simulink model "fangzheng"  (R2023b)
settings: Solver=ode45  StartTime=0.0  StopTime=1.5  RelTol=1e-6
InitFcn:
  | Rf=0.05;Lf=2e-3;Cf=50e-6;fn=50;w0=2*fn*pi;
  | UB=3e3;SB=1e6;IB=SB/(sqrt(3)*UB);
  | Xf=Lf*w0;Z=sqrt((Rf^2+Xf^2));
  | J=3;D=2e4/w0*0;kf=0.9e4/w0;
  | K=230*380/Xf;
  | P=10;I=12e3;
  | Jw=8e4;
  | Pi=1;Pp=0;P2 =1000;
  | U5=30;
  | U7=15;
undefined symbols (not defined in the file): sigbuilder_block
libraries: slpidlib x5, spsThreePhaseSeriesRLCBranchLib x4, spsThreePhaseBreakerLib x3, spsabctodq0Lib x3, simulink x3, spsThreePhaseVIMeasurementLib x3, spsControlledVoltageSourceLib x3, spsThreePhaseSeriesRLCLoadLib x2, spsDCVoltageSourceLib x1, spsUniversalBridgeLib x1, spsPWMGenerator2LevelLib x1, spsdq0toabcLib x1
settings Model: SimulationMode=accelerator  Creator=lenovo  LastModifiedBy=Administrator
settings SolverCC: ZeroCrossAlgorithm=Adaptive  AlgebraicLoopSolver=TrustRegion
settings DataIOCC: SaveFormat=StructureWithTime  ReturnWorkspaceOutputs=off
settings OptimizationCC: DefaultParameterBehavior=Inlined  EnhancedBackFolding=on  PassReuseOutputArgsAs=Individual arguments  ZeroExternalMemoryAtStartup=off  ZeroInternalMemoryAtStartup=off  AccelVerboseBuild=on  OptimizeBlockOrder=speed  DifferentSizesBufferReuse=on  OptimizationCustomize=off  EfficientTunableParamExpr=on
settings DebuggingCC: IgnoredZcDiagnostic=none  ParameterTunabilityLossMsg=error  UnconnectedInputMsg=warning  UnconnectedOutputMsg=warning  UnconnectedLineMsg=warning  ArithmeticOperatorsInVariantConditions=warning
settings ModelReferenceCC: EnableRefExpFcnMdlSchedulingChecks=on
settings SFSimCC: MATLABDynamicMemAlloc=off  CustomCodeUndefinedFunction=UseInterfaceOnly
settings RTWCC: Description=Embedded Coder  SystemTargetFile=ert.tlc  TemplateMakefile=ert_default_tmf
settings CodeAppCC: ForceParamTrailComments=on  IgnoreCustomStorageClasses=off  OperatorAnnotations=on  SimulinkDataObjDesc=on  SFDataObjDesc=on  InsertBlockDesc=on
settings ERTTargetCC: TargetLangStandard=C99 (ISO)  GenerateSampleERTMain=on  InlinedParameterPlacement=NonHierarchical  ERTCustomFileTemplate=example_file_process.tlc

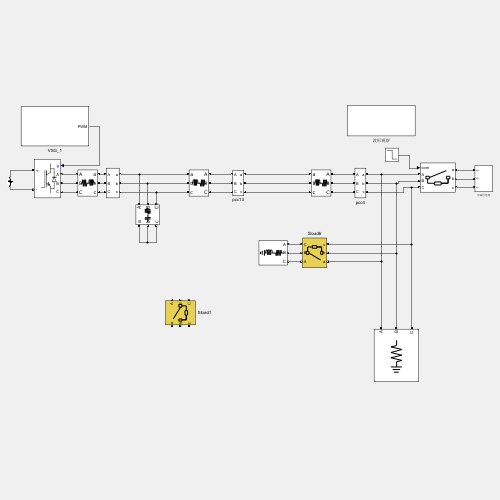
[thumbnail: Simulink's stored preview of the top-level diagram]
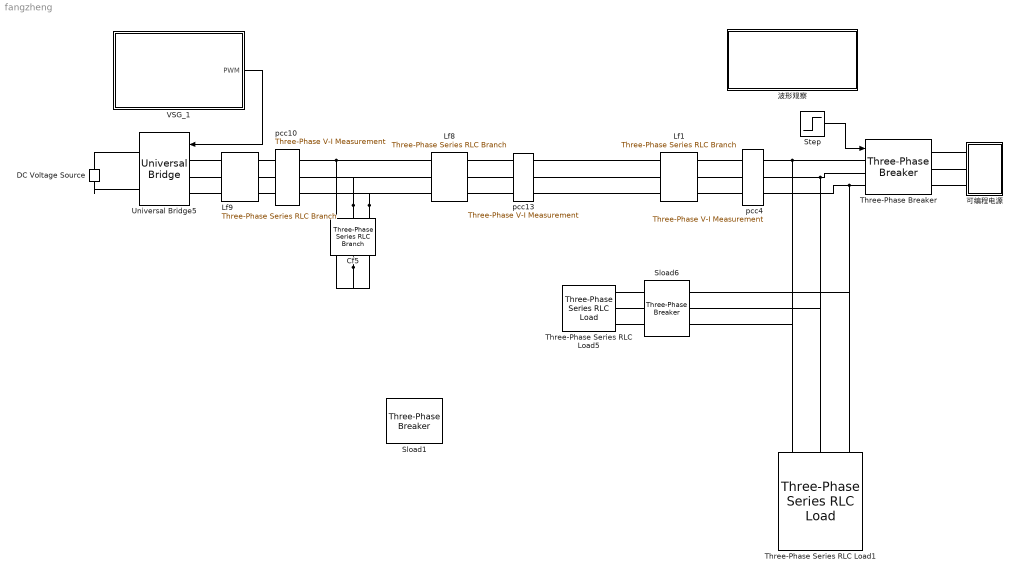
== system fangzheng ==
  " Lf1" : spsThreePhaseSeriesRLCBranchLib/Three-Phase Series RLC Branch  LConnTagsString=A|B|C  RConnTagsString=A|B|C  BranchType=RL  Resistance=0.1  Inductance=0.0002  Capacitance=0  Measurements=None
  " Lf8" : spsThreePhaseSeriesRLCBranchLib/Three-Phase Series RLC Branch  LConnTagsString=A|B|C  RConnTagsString=A|B|C  BranchType=RL  Resistance=0.02  Inductance=0.004  Capacitance=0  Measurements=None
  " Lf9" : spsThreePhaseSeriesRLCBranchLib/Three-Phase Series RLC Branch  LConnTagsString=A|B|C  RConnTagsString=A|B|C  BranchType=RL  Resistance=0.1  Inductance=0.005  Capacitance=0  Measurements=None
  Cf5 : spsThreePhaseSeriesRLCBranchLib/Three-Phase Series RLC Branch  LConnTagsString=A|B|C  RConnTagsString=A|B|C  BranchType=RC  Resistance=0.5  Inductance=4e-3  Capacitance=3e-5  Measurements=None
  DC Voltage Source : spsDCVoltageSourceLib/DC Voltage Source  Amplitude=800  Measurements=None
  Sload1 : spsThreePhaseBreakerLib/Three-Phase Breaker  InitialState=open  SwitchA=on  SwitchB=on  SwitchC=on  SwitchTimes=[1.0]  External=off  BreakerResistance=0.0001  SnubberResistance=1e6  SnubberCapacitance=inf  Measurements=None
  Sload6 : spsThreePhaseBreakerLib/Three-Phase Breaker  InitialState=open  SwitchA=on  SwitchB=on  SwitchC=on  SwitchTimes=[1.2]  External=off  BreakerResistance=0.0001  SnubberResistance=1e6  SnubberCapacitance=inf  Measurements=None
  Step : Step  Before=1  After=0  SampleTime=0
  Three-Phase Series RLC Load1 : spsThreePhaseSeriesRLCLoadLib/Three-Phase Series RLC Load  LConnTagsString=A|B|C  Configuration=Y (grounded)  NominalVoltage=380  Vabc=[1e3 1e3 1e3]  Vabcp=[1e3 1e3 1e3]  NominalFrequency=50  UnbalancedPower=off  ActivePower=15e3  InductivePower=0  CapacitivePower=0  Pabc=[10e3 9e3 11e3]  QLabc=[100 90 110]  QCabc=[100 90 110]  Pabcp=[10e3 9e3 11e3]  QLabcp=[100 90 110]  QCabcp=[100 90 110]  Measurements=None  LoadType=constant Z
  Three-Phase Series RLC Load5 : spsThreePhaseSeriesRLCLoadLib/Three-Phase Series RLC Load  LConnTagsString=A|B|C  Configuration=Y (grounded)  NominalVoltage=380  Vabc=[1e3 1e3 1e3]  Vabcp=[1e3 1e3 1e3]  NominalFrequency=50  UnbalancedPower=off  ActivePower=15e3  InductivePower=6e3  CapacitivePower=0  Pabc=[10e3 9e3 11e3]  QLabc=[100 90 110]  QCabc=[100 90 110]  Pabcp=[10e3 9e3 11e3]  QLabcp=[100 90 110]  QCabcp=[100 90 110]  Measurements=None  LoadType=constant Z
  Three-Phase Breaker : spsThreePhaseBreakerLib/Three-Phase Breaker  InitialState=open  SwitchA=on  SwitchB=on  SwitchC=on  SwitchTimes="[1/60  5/60]"  External=on  BreakerResistance=0.01  SnubberResistance=1e6  SnubberCapacitance=inf  Measurements=None
  Universal Bridge5 : spsUniversalBridgeLib/Universal Bridge  Arms=3  SnubberResistance=1e5  SnubberCapacitance=inf  Device=IGBT / Diodes  Ron=1e-5  Lon=0  ForwardVoltages=[0.05 0.05]  ForwardVoltage=0  GTOparameters=[ 10e-6 , 20e-6 ]  IGBTparameters=[ 1e-6 , 2e-6 ]  Measurements=None  Measurements_2=None  converterType=Rectifier
  VSG_1 : Subsystem
  pcc10 : spsThreePhaseVIMeasurementLib/Three-Phase V-I Measurement  VoltageMeasurement=phase-to-ground  SetLabelV=on  LabelV=Vo_1  Vpu=off  VpuLL=off  CurrentMeasurement=yes  SetLabelI=on  LabelI=IL_1  Ipu=off  Pbase=1e6  Vbase=6.6e3/sqrt(3)  OutputType=Magnitude  PhasorSimulation=off  PSBequivalent=0
  pcc13 : spsThreePhaseVIMeasurementLib/Three-Phase V-I Measurement  VoltageMeasurement=phase-to-ground  SetLabelV=on  LabelV=Vabc_pcc_1  Vpu=off  VpuLL=off  CurrentMeasurement=yes  SetLabelI=on  LabelI=Iabc_pcc_1  Ipu=off  Pbase=1e6  Vbase=6.6e3/sqrt(3)  OutputType=Magnitude  PhasorSimulation=off  PSBequivalent=0
  pcc4 : spsThreePhaseVIMeasurementLib/Three-Phase V-I Measurement  VoltageMeasurement=phase-to-ground  SetLabelV=on  LabelV=Vg  Vpu=off  VpuLL=off  CurrentMeasurement=yes  SetLabelI=on  LabelI=Ig  Ipu=off  Pbase=1e6  Vbase=6.6e3/sqrt(3)  OutputType=Magnitude  PhasorSimulation=off  PSBequivalent=0
  可编程电源 : Subsystem
  波形观察 : Subsystem
  wires:
  VSG_1/1(PWM) -> Universal Bridge5/1
  Step/1 -> Three-Phase Breaker/1
  connections:
  Cf5/RConn2 -- Cf5/RConn3 -- Cf5/RConn1
  " Lf9"/LConn3 -- Universal Bridge5/LConn3
  " Lf9"/LConn1 -- Universal Bridge5/LConn1
  " Lf9"/LConn2 -- Universal Bridge5/LConn2
  " Lf8"/RConn1 -- pcc10/RConn1 -- Cf5/LConn1
  Cf5/LConn3 -- pcc10/RConn3 -- " Lf8"/RConn3
  Cf5/LConn2 -- pcc10/RConn2 -- " Lf8"/RConn2
  " Lf1"/LConn2 -- pcc4/LConn2
  pcc4/LConn3 -- " Lf1"/LConn3
  pcc4/LConn1 -- " Lf1"/LConn1
  " Lf1"/RConn1 -- pcc13/RConn1
  " Lf1"/RConn2 -- pcc13/RConn2
  " Lf1"/RConn3 -- pcc13/RConn3
  " Lf8"/LConn1 -- pcc13/LConn1
  " Lf8"/LConn2 -- pcc13/LConn2
  " Lf8"/LConn3 -- pcc13/LConn3
  DC Voltage Source/RConn1 -- Universal Bridge5/RConn1
  DC Voltage Source/LConn1 -- Universal Bridge5/RConn2
  " Lf9"/RConn1 -- pcc10/LConn1
  " Lf9"/RConn2 -- pcc10/LConn2
  " Lf9"/RConn3 -- pcc10/LConn3
  Three-Phase Breaker/RConn1 -- 可编程电源/RConn1
  Three-Phase Breaker/RConn2 -- 可编程电源/RConn2
  Three-Phase Breaker/RConn3 -- 可编程电源/RConn3
  Sload6/LConn3 -- Three-Phase Series RLC Load5/LConn1
  Sload6/LConn2 -- Three-Phase Series RLC Load5/LConn2
  Sload6/LConn1 -- Three-Phase Series RLC Load5/LConn3
  Three-Phase Breaker/LConn1 -- Three-Phase Series RLC Load1/LConn1 -- Sload6/RConn1 -- pcc4/RConn1
  pcc4/RConn2 -- Three-Phase Series RLC Load1/LConn2 -- Sload6/RConn2 -- Three-Phase Breaker/LConn2
  Three-Phase Breaker/LConn3 -- Sload6/RConn3 -- Three-Phase Series RLC Load1/LConn3 -- pcc4/RConn3

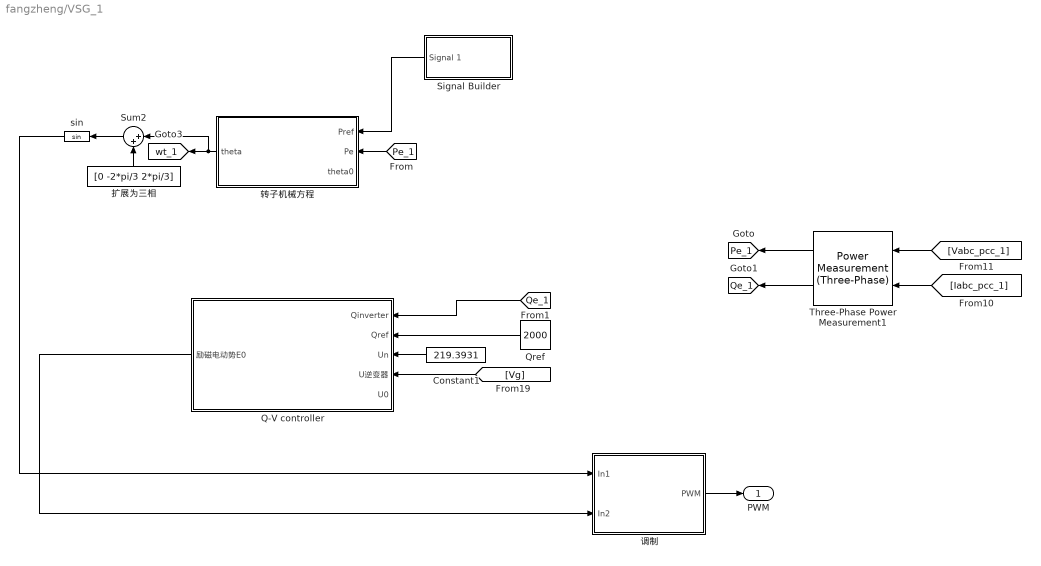
== system fangzheng/VSG_1 ==
  " 调制" : Subsystem
  Constant1 : Constant  Value=219.3931
  Q-V controller : Subsystem
  Qref : Constant  Value=2000
  Signal Builder : Subsystem  Tag=STV Subsys  LoadFcn=sigbuilder_block('load');  StartFcn=sigbuilder_block('start');  StopFcn=sigbuilder_block('stop');  ClipboardFcn=sigbuilder_block('clipboard');  mask(Sigbuilder block){tuvar=[0:10]}
      mask help: Simulink:masks:SigbuilderBlock_MD
      mask init:
      | if ~strcmp(get_param(bdroot(gcbh),'SimulationStatus'),'stopped') tuvar = sigbuilder_block('maskInit'); end
      settings: CopyFcn=sigbuilder_block('copy');  DeleteFcn=sigbuilder_block('delete');  ModelCloseFcn=sigbuilder_block('modelClose');  PreSaveFcn=sigbuilder_block('preSave');  PauseFcn=sigbuilder_block('pause');  ContinueFcn=sigbuilder_block('continue');  NameChangeFcn=sigbuilder_block('namechange');  OpenFcn=sigbuilder_block('open',[4.875 36 1430.25 685.125 ]);  CloseFcn=sigbuilder_block('close');
      mask Display: plot(0, 0, 100, 100,[2, 2, 32, 32, 2], [68, 8, 8, 68, 68],[32, 2], [38, 38], [32, 19, 2],[53, 60, 44], [32, 17, 17, 2],[16, 16, 31, 31]);txt = getActiveGroup(gcbh);text(2, 100, txt,'verticalAlignment', 'top');
  Sum2 : Sum  Inputs=|++
  Three-Phase Power Measurement1 : eePowerMeasurement/Power Measurement (Three-Phase)  LabelModeActiveChoice=Continuous  F=50  K=[1]  Seq=Positive  Ts=0
  sin : Trigonometry
  扩展为三相 : Constant  Value=[0 -2*pi/3 2*pi/3]
  转子机械方程 : Subsystem
  PWM : Outport
  tag scope: Pe_1=global, Qe_1=global, wt_1=global
  wires:
  扩展为三相/1 -> Sum2/2
  Three-Phase Power Measurement1/1 -> [Pe_1]
  [Iabc_pcc_1] -> Three-Phase Power Measurement1/2
  Qref/1 -> Q-V controller/2(Qref)
  [Vg] -> Q-V controller/4(U逆变器)
  [Vabc_pcc_1] -> Three-Phase Power Measurement1/1
  转子机械方程/1(theta) -> Sum2/1, [wt_1]
  Three-Phase Power Measurement1/2 -> [Qe_1]
  Constant1/1 -> Q-V controller/3(Un)
  Sum2/1 -> sin/1
  Signal Builder/1(Signal 1) -> 转子机械方程/1(Pref)
  sin/1 -> " 调制"/1(In1)
  Q-V controller/1(励磁电动势E0) -> " 调制"/2(In2)
  " 调制"/1(PWM) -> PWM/1
  [Pe_1] -> 转子机械方程/2(Pe)
  [Qe_1] -> Q-V controller/1(Qinverter)

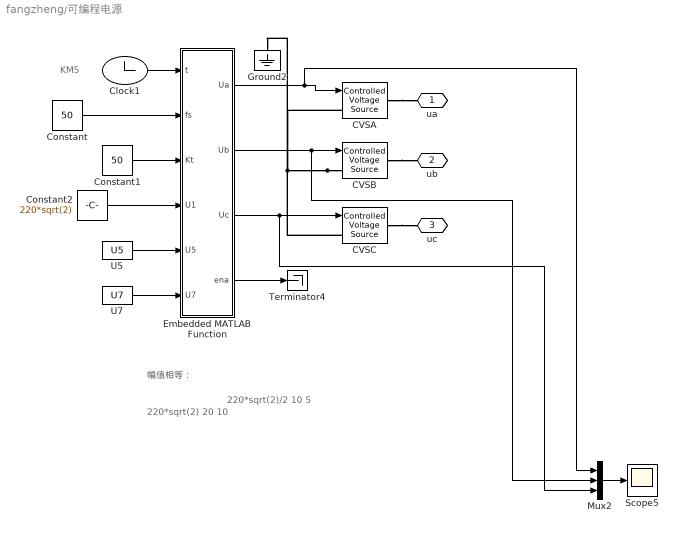
== system fangzheng/可编程电源 ==
  note: KM5
  note: 幅值相等：
  note: 220*sqrt(2)
      | 20
      | 10
  note: 220*sqrt(2)/2
      | 10
      | 5
  CVSA : spsControlledVoltageSourceLib/Controlled Voltage Source  Initialize=on  Source_Type=AC  Amplitude=0  Phase=0  Frequency=0  Measurements=None
  CVSB : spsControlledVoltageSourceLib/Controlled Voltage Source  Initialize=on  Source_Type=AC  Amplitude=0  Phase=0  Frequency=0  Measurements=None
  CVSC : spsControlledVoltageSourceLib/Controlled Voltage Source  Initialize=on  Source_Type=AC  Amplitude=0  Phase=0  Frequency=0  Measurements=None
  Clock1 : Clock
  Constant : Constant  Value=50
  Constant1 : Constant  Value=50
  Constant2 : Constant  Value=220*sqrt(2)
  Embedded MATLAB Function : MATLAB Function  TreatAsAtomicUnit=on
  Ground2 : spsGroundLib/Ground  LConnTagsString=a
  Mux2 : Mux  Inputs=3
  Scope5 : Scope
  Terminator4 : Terminator
  U5 : Constant  Value=U5
  U7 : Constant  Value=U7
  ua : PMIOPort  Side=Right
  ub : PMIOPort  Port=2  Side=Right
  uc : PMIOPort  Port=3  Side=Right
  wires:
  Clock1/1 -> Embedded MATLAB Function/1(t)
  U5/1 -> Embedded MATLAB Function/5(U5)
  Embedded MATLAB Function/3(Uc) -> Mux2/3, CVSC/1
  U7/1 -> Embedded MATLAB Function/6(U7)
  Embedded MATLAB Function/4(ena) -> Terminator4/1
  Constant1/1 -> Embedded MATLAB Function/3(Kt)
  Constant/1 -> Embedded MATLAB Function/2(fs)
  Embedded MATLAB Function/2(Ub) -> Mux2/2, CVSB/1
  Mux2/1 -> Scope5/1
  Embedded MATLAB Function/1(Ua) -> Mux2/1, CVSA/1
  Constant2/1 -> Embedded MATLAB Function/4(U1)
  connections:
  CVSC/RConn1 -- uc/RConn1
  CVSB/RConn1 -- ub/RConn1
  CVSA/RConn1 -- ua/RConn1
  CVSB/LConn1 -- Ground2/LConn1 -- CVSA/LConn1 -- CVSC/LConn1

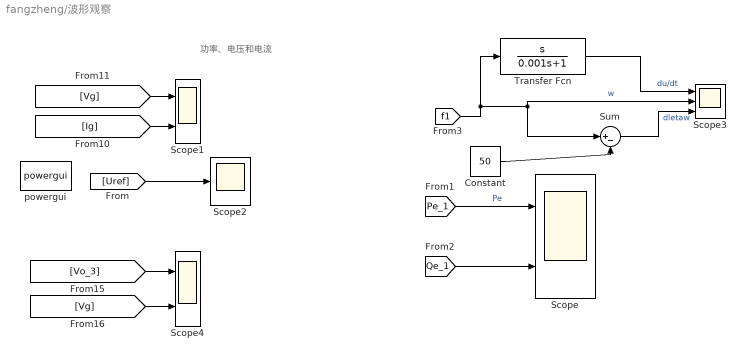
== system fangzheng/波形观察 ==
  note: 功率、电压和电流
  Constant : Constant  Value=50
  Scope : Scope  NumInputPorts=2
  Scope1 : Scope  NumInputPorts=2
  Scope2 : Scope
  Scope3 : Scope  NumInputPorts=3
  Scope4 : Scope  NumInputPorts=2
  Sum : Sum  Inputs=|+-
  Transfer Fcn : TransferFcn  Numerator=[1 0]  Denominator=[0.001 1]
  powergui : sps_lib/powergui  Priority=1  SimulationMode=Discrete  SampleTime=1e-6  frequency=60  Iterations=50  frequencyindice=0  Pbase=100e6  ErrMax=1e-4  UnitsV=kV  UnitsW=MW  buscounter=0  FunctionMessages=off  echomessages=off  EnableUseOfTLC=off  CurrentSourceSwitches=off  DisableSnubberDevices=off  DisableRonSwitches=off  DisableVfSwitches=off  DisplayEquations=off  AutomaticDiscreteSolvers=off  SolverType=Tustin/Backward Euler (TBE)  Interpol=off  ExternalGateDelay=off  methode=off  Ts=100  x0status=blocks  SPID=on  SwTol=0  HookPort=off  NonlinearTolerance=1e-4  nMaxIteration=100  ContinueOnMaxIteration=off  RestoreLinks=warning  ResistiveCurrentMeasurement=off  Frange=[0:2:500]  Ylog=off  Xlog=on  ShowGrid=off  save=off  variable=ZData  structure=logsout  ZoomFFT=off  StartTime=0.5  cycles=10  DisplayStyle=1  fundamental=50  FreqAxis=off  MaxFrequency=1000  frequencyindicesteady=1  RmsSteady=1  display=off
  wires:
  [Vg] -> Scope1/1
  [Qe_1] -> Scope/2
  [Pe_1] -> Scope/1  "Pe"
  [Ig] -> Scope1/2
  [Uref] -> Scope2/1
  [f1] -> Sum/1, Scope3/2, Transfer Fcn/1  "w"
  [Vo_3] -> Scope4/1
  [Vg] -> Scope4/2
  Transfer Fcn/1 -> Scope3/1  "du/dt"
  Constant/1 -> Sum/2
  Sum/1 -> Scope3/3  "dletaw"

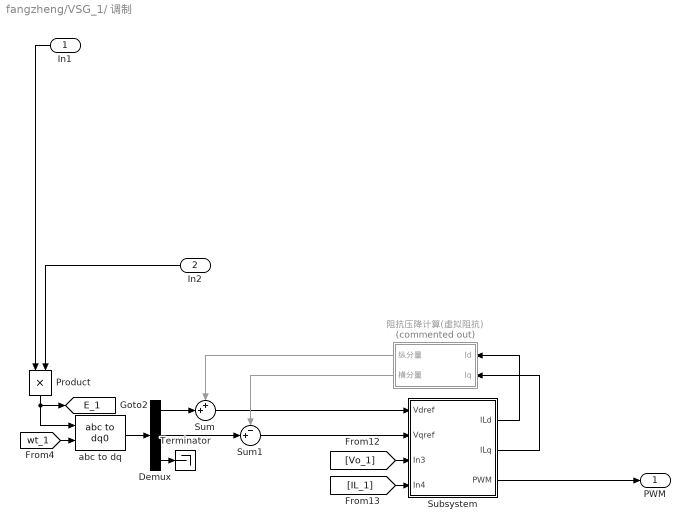
== system fangzheng/VSG_1/ 调制 ==
  In1 : Inport
  In2 : Inport  Port=2
  Demux : Demux  Outputs=3
  Product : Product
  Subsystem : Subsystem
  Sum : Sum  Inputs=++|
  Sum1 : Sum  Inputs=-+|
  Terminator : Terminator
  abc to dq : spsabctodq0Lib/abc to dq0  Alignment=90 degrees behind phase A axis
  阻抗压降计算(虚拟阻抗) : Subsystem  Commented=on
  PWM : Outport
  tag scope: E_1=global
  wires:
  [Vo_1] -> Subsystem/3(In3)
  Demux/2 -> Sum1/2
  Sum/1 -> Subsystem/1(Vdref)
  [IL_1] -> Subsystem/4(In4)
  abc to dq/1 -> Demux/1
  Subsystem/1(ILd) -> 阻抗压降计算(虚拟阻抗)/1(Id)
  Demux/1 -> Sum/2
  阻抗压降计算(虚拟阻抗)/1(纵分量) -> Sum/1
  Demux/3 -> Terminator/1
  Sum1/1 -> Subsystem/2(Vqref)
  Product/1 -> [E_1], abc to dq/1
  Subsystem/2(ILq) -> 阻抗压降计算(虚拟阻抗)/2(Iq)
  阻抗压降计算(虚拟阻抗)/2(横分量) -> Sum1/1
  Subsystem/3(PWM) -> PWM/1
  [wt_1] -> abc to dq/2
  In1/1 -> Product/1
  In2/1 -> Product/2

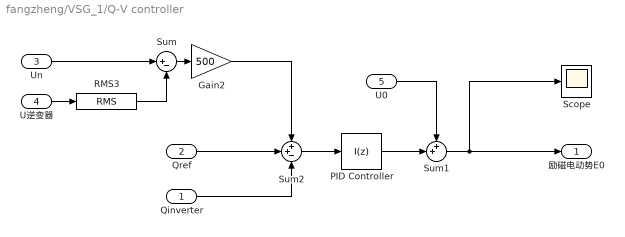
== system fangzheng/VSG_1/Q-V controller ==
  Qinverter : Inport
  Qref : Inport  Port=2
  Un : Inport  Port=3
  U逆变器 : Inport  Port=4
  U0 : Inport  Port=5
  Gain2 : Gain  Gain=500
  PID Controller : slpidlib/PID Controller  Controller=I  Form=Parallel  TimeDomain=Discrete-time  UseExternalTs=off  SampleTime=-1  IntegratorMethod=Forward Euler  FilterMethod=Forward Euler  ControllerParametersSource=internal  P=0.0000001  I=1.1547e-5*5  UseKiTs=off  D=0  N=100  UseFilter=on  TunerSelectOption=Transfer Function Based (PID Tuner App)  InitialConditionSource=internal  InitialConditionForIntegrator=0  InitialConditionForFilter=0  DifferentiatorICPrevScaledInput=0  ExternalReset=none  TrackingMode=off  Kt=1  LimitOutput=off  SatLimitsSource=internal  UpperSaturationLimit=inf  LowerSaturationLimit=-inf  LinearizeAsGain=on  AntiWindupMode=none  Kb=1  LimitIntegrator=off  UpperIntegratorSaturationLimit=inf  LowerIntegratorSaturationLimit=-inf  POutMin=[]  POutMax=[]  IOutMin=[]  IOutMax=[]  DOutMin=[]  DOutMax=[]  NOutMin=[]  NOutMax=[]  SumOutMin=[]  SumOutMax=[]  SaturationOutMin=[]  SaturationOutMax=[]  PParamMin=[]  PParamMax=[]  IParamMin=[]  IParamMax=[]  DParamMin=[]  DParamMax=[]  NParamMin=[]  NParamMax=[]  KbParamMin=[]  KbParamMax=[]  KtParamMin=[]  KtParamMax=[]  KbOutMin=[]  KbOutMax=[]  KtOutMin=[]  KtOutMax=[]  IntegratorOutMin=[]  IntegratorOutMax=[]  FilterOutMin=[]  FilterOutMax=[]  SumI1OutMin=[]  SumI1OutMax=[]  SumI2OutMin=[]  SumI2OutMax=[]  SumI3OutMin=[]  SumI3OutMax=[]  SumI4OutMin=[]  SumI4OutMax=[]  SumDOutMin=[]  SumDOutMax=[]  DifferentiatorOutMin=[]  DifferentiatorOutMax=[]  FilterDiffOutCoefMin=[]  FilterDiffOutCoefMax=[]  ReciprocalOutMin=[]  ReciprocalOutMax=[]  SumDenOutMin=[]  SumDenOutMax=[]  SumNumOutMin=[]  SumNumOutMax=[]  DivideOutMin=[]  DivideOutMax=[]  UdiffTsProdOutMin=[]  UdiffTsProdOutMax=[]  NTsProdOutMin=[]  NTsProdOutMax=[]  UintegralTsProdOutMin=[]  UintegralTsProdOutMax=[]  UngainTsProdOutMin=[]  UngainTsProdOutMax=[]  ClampingZeroOutDataTypeStr=Inherit: Inherit via back propagation  ClampingZeroOutMin=[]  ClampingZeroOutMax=[]  FilterDenConstantOutDataTypeStr=Inherit: Inherit via back propagation  FilterDenConstantOutMin=[]  FilterDenConstantOutMax=[]  PCopyOutDataTypeStr=Inherit: Inherit via back propagation  PCopyOutMin=[]  PCopyOutMax=[]  NCopyOutDataTypeStr=Inherit: Inherit via back propagation  NCopyOutMin=[]  NCopyOutMax=[]  IntegratorContinuousStateAttributes=''  IntegratorStateMustResolveToSignalObject=off  IntegratorRTWStateStorageClass=Auto  FilterContinuousStateAttributes=''  FilterStateMustResolveToSignalObject=off  FilterRTWStateStorageClass=Auto  ParallelPVariant=Disabled  IdealPVariant=Disabled  IVariant=InternalParameters  DVariant=Disabled  IntegratorVariant=Discrete  SatVariant=Disabled  AWVariant=Passthrough  PCopyVariant=Disabled  TRVariant=Disabled  FdbkBlocksVariant=Forward  IdealPFdbkVariant=Disabled  SatFdbkVariant=Disabled  DerivativeFilterVariant=Disabled  NVariant=Disabled  NCopyVariant=Disabled_SignalSpec  FilterICVariant=Disabled  IntegratorICVariant=InternalICs  ExternalResetVariant=Disabled  TRSumVariant=Passthrough  SumFdbkVariant=Disabled  SumVariant=Passthrough_I  TsampFilterVariant=InternalTs  TsampNgainVariant=Passthrough  TsampIntegralVariant=Disabled_SignalSpec  ExternalSaturationOutDataTypeStr=Inherit: Same as second input
  RMS3 : dspstat3/RMS  run=off  directionMode=Each column  dimension=1  InputProcessing=Columns as channels (frame based)  reset_popup=None
  Scope : Scope
  Sum : Sum  Inputs=|+-
  Sum1 : Sum  Inputs=++|
  Sum2 : Sum  Inputs=++-
  励磁电动势E0 : Outport
  wires:
  Qinverter/1 -> Sum2/3
  Qref/1 -> Sum2/2
  Un/1 -> Sum/1
  U逆变器/1 -> RMS3/1
  Gain2/1 -> Sum2/1
  Sum/1 -> Gain2/1
  RMS3/1 -> Sum/2
  Sum2/1 -> PID Controller/1
  U0/1 -> Sum1/1
  Sum1/1 -> 励磁电动势E0/1, Scope/1
  PID Controller/1 -> Sum1/2

== system fangzheng/VSG_1/Signal Builder ==
  Demux : Demux  Tag=STV Demux  Outputs=1
      settings: DisplayOption=none
  FromWs : FromWorkspace  Tag=STV FromWs  VariableName=tuvar
      SigBuilderData=|
      | common.afterFinalStr = 'Extrapolate'
      | common.sampleTime = 0
      | dataSet.timeRange = [0 10]
      | dataSet.name = 'Group 1'
      | sbobj.Groups.Name = 'Group 1'
      | sbobj.Groups.Signals.Name = 'Signal 1'
      | sbobj.Groups.Signals.XData = [0 0.5 0.5 2 2 3.93 3.93 6 6 10]
      | sbobj.Groups.Signals.YData = [0 0 15700 15700 30100 30100 0 0 -0.2 -0.2]
  Signal 1 : Outport  Tag=STV Outport  VectorParamsAs1DForOutWhenUnconnected=off
  wires:
  FromWs/1 -> Demux/1
  Demux/1 -> Signal 1/1

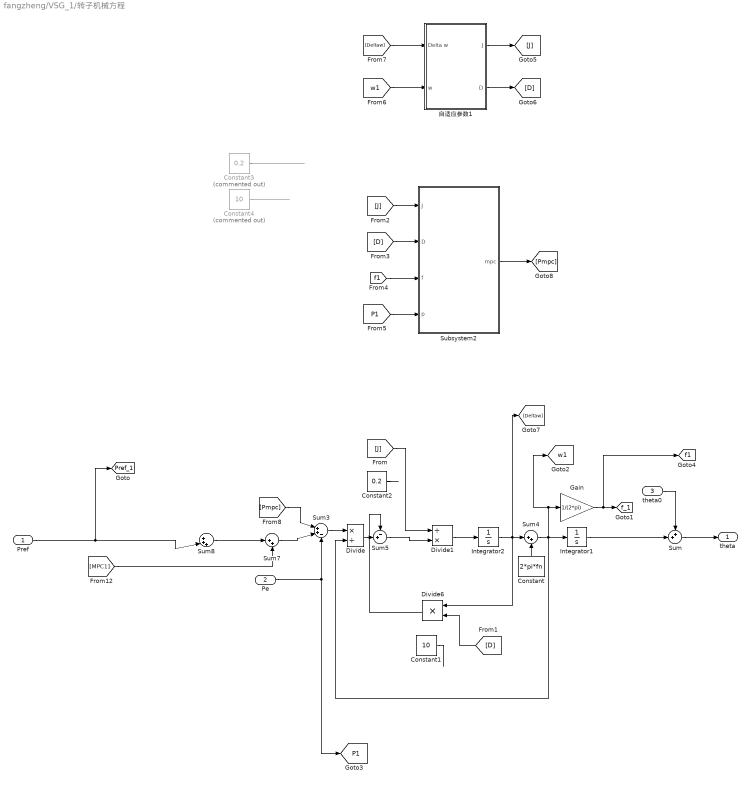
== system fangzheng/VSG_1/转子机械方程 ==
  Pref : Inport
  Pe : Inport  Port=2
  theta0 : Inport  Port=3
  Constant : Constant  Value=2*pi*fn
  Constant1 : Constant  Value=10
  Constant2 : Constant  Value=0.2
  Constant3 : Constant  Commented=on  Value=0.2
  Constant4 : Constant  Commented=on  Value=10
  Divide : Product  Inputs=*/
  Divide1 : Product  Inputs=/*
  Divide6 : Product  Inputs=**
  Gain : Gain  Gain=1/(2*pi)
  Integrator1 : Integrator
  Integrator2 : Integrator
  Subsystem2 : Subsystem
  Sum : Sum  Inputs=++|
  Sum3 : Sum  Inputs=|++-
  Sum4 : Sum  Inputs=|++
  Sum5 : Sum  Inputs=-+|
  Sum7 : Sum  Inputs=|++
  Sum8 : Sum  Inputs=|+++
  自适应参数1 : Subsystem
  theta : Outport
  tag scope: P1=global, Pref_1=global, f1=global, f_1=global, w1=global
  wires:
  Constant/1 -> Sum4/2
  Divide/1 -> Sum5/2
  Sum3/1 -> Divide/1
  Divide1/1 -> Integrator2/1
  theta0/1 -> Sum/1
  Sum/1 -> theta/1
  Integrator1/1 -> Sum/2
  Subsystem2/1(mpc) -> [Pmpc]
  Pref/1 -> Sum8/2, [Pref_1]
  Sum8/1 -> Sum7/1
  Gain/1 -> [f1], [f_1]
  Sum7/1 -> Sum3/2
  Pe/1 -> Sum3/3, [P1]
  [MPC1] -> Sum7/2
  Divide6/1 -> Sum5/1
  [D] -> Divide6/2
  Sum5/1 -> Divide1/2
  Constant2/1 -> ?
  自适应参数1/2(D) -> [D]
  Sum4/1 -> Divide/2, Integrator1/1, [w1], Gain/1
  Integrator2/1 -> [Deltaw], Divide6/1, Sum4/1
  自适应参数1/1(J) -> [J]
  Constant3/1 -> ?
  Constant4/1 -> ?
  [J] -> Divide1/1
  [J] -> Subsystem2/1(J)
  [D] -> Subsystem2/2(D)
  Constant1/1 -> ?
  [f1] -> Subsystem2/3(f)
  [P1] -> Subsystem2/4(p)
  [w1] -> 自适应参数1/2(w)
  [Deltaw] -> 自适应参数1/1(Delta w)
  [Pmpc] -> Sum3/1

== system fangzheng/VSG_1/ 调制/Subsystem ==
  Vdref : Inport
  Vqref : Inport  Port=2
  In3 : Inport  Port=3
  In4 : Inport  Port=4
  Gain5 : Gain  Gain=1/(SB/(sqrt(3)*UB))
  Gain6 : Gain  Gain=sqrt(3)/UB
  abc2dq0 : Subsystem
  电压电流双闭环 : Subsystem
  ILd : Outport
  ILq : Outport  Port=2
  PWM : Outport  Port=3
  wires:
  Vqref/1 -> 电压电流双闭环/2(Vqref)
  In4/1 -> Gain5/1
  abc2dq0/1(Vd) -> 电压电流双闭环/3(Vd)
  abc2dq0/2(Vq) -> 电压电流双闭环/4(Vq)
  abc2dq0/3(ILd) -> 电压电流双闭环/5(ILd), ILd/1
  Gain5/1 -> abc2dq0/2(Iabc)
  Gain6/1 -> abc2dq0/1(Vabc)
  abc2dq0/4(ILq) -> 电压电流双闭环/6(ILq), ILq/1
  电压电流双闭环/1(PWM) -> PWM/1
  Vdref/1 -> 电压电流双闭环/1(Vdref)
  In3/1 -> Gain6/1

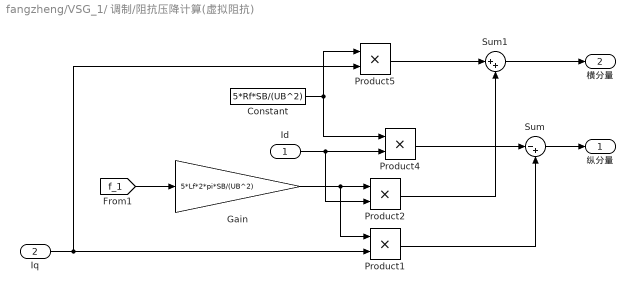
== system fangzheng/VSG_1/ 调制/阻抗压降计算(虚拟阻抗) ==
  Id : Inport
  Iq : Inport  Port=2
  Constant : Constant  Value=5*Rf*SB/(UB^2)
  Gain : Gain  Gain=5*Lf*2*pi*SB/(UB^2)
  Product{1..2,4..5} (4 alike) : Product
  Sum : Sum  Inputs=|-+
  Sum1 : Sum  Inputs=|++
  纵分量 : Outport
  横分量 : Outport  Port=2
  wires:
  Product2/1 -> Sum1/2
  Sum1/1 -> 横分量/1
  Product5/1 -> Sum1/1
  Sum/1 -> 纵分量/1
  Product1/1 -> Sum/2
  Product4/1 -> Sum/1
  Gain/1 -> Product1/1, Product2/1
  Iq/1 -> Product5/2, Product1/2
  [f_1] -> Gain/1
  Constant/1 -> Product5/1, Product4/1
  Id/1 -> Product2/2, Product4/2

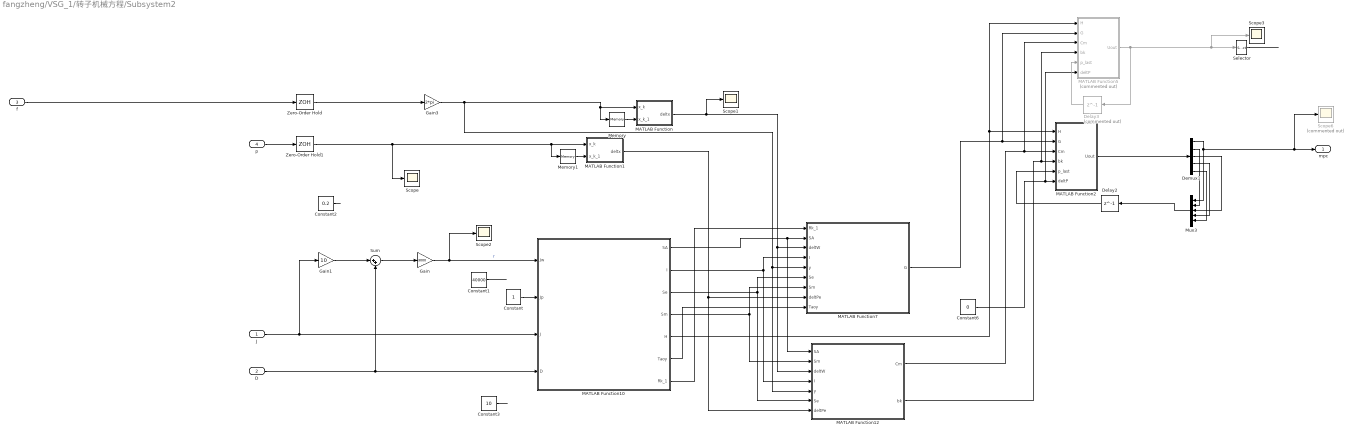
== system fangzheng/VSG_1/转子机械方程/Subsystem2 ==
  J : Inport
  D : Inport  Port=2
  f : Inport  Port=3
  p : Inport  Port=4
  Constant : Constant
  Constant1 : Constant  Value=40000
  Constant2 : Constant  Value=0.2
  Constant3 : Constant  Value=10
  Constant6 : Constant  Value=0
  Delay2 : Delay  DelayLength=1  InitialCondition=zeros(5,1)
  Delay3 : Delay  Commented=on  DelayLength=1  InitialCondition=zeros(5,1)
  Demux1 : Demux  Outputs=5
  Gain : Gain  Gain=3000
  Gain1 : Gain  Gain=10
  Gain3 : Gain  Gain=2*pi
  MATLAB Function : MATLAB Function  TreatAsAtomicUnit=on
  MATLAB Function1 : MATLAB Function  TreatAsAtomicUnit=on
  MATLAB Function10 : MATLAB Function  TreatAsAtomicUnit=on
  MATLAB Function12 : MATLAB Function  TreatAsAtomicUnit=on
  MATLAB Function2 : MATLAB Function  TreatAsAtomicUnit=on
  MATLAB Function5 : MATLAB Function  Commented=on  TreatAsAtomicUnit=on
  MATLAB Function7 : MATLAB Function  TreatAsAtomicUnit=on
  Memory : Memory
  Memory1 : Memory
  Mux3 : Mux  Inputs=5
  Scope{,1..3} (4 alike) : Scope
  Scope6 : Scope  Commented=on
  Selector : Selector  InputPortWidth=5  IndexOptions=Index vector (dialog)  Indices=[1]  OutputSizes=1
  Sum : Sum  Inputs=|++
  Zero-Order Hold : ZeroOrderHold  SampleTime=2e-5
  Zero-Order Hold1 : ZeroOrderHold  SampleTime=2e-5
  mpc : Outport
  wires:
  Demux1/4 -> Mux3/4
  Memory/1 -> MATLAB Function/2(x_k_1)
  Demux1/2 -> Mux3/2
  MATLAB Function2/1(Uout) -> Demux1/1
  MATLAB Function1/1(deltx) -> MATLAB Function7/8(deltPe), MATLAB Function12/7(deltPe)
  MATLAB Function10/3(Se) -> MATLAB Function7/6(Se), MATLAB Function12/6(Se)
  MATLAB Function10/1(SA) -> MATLAB Function12/1(SA), MATLAB Function7/2(SA)
  MATLAB Function10/6(Taoy) -> MATLAB Function7/9(Taoy)
  MATLAB Function7/1(G) -> MATLAB Function5/2(G), MATLAB Function2/2(G)
  Demux1/5 -> Mux3/5
  Demux1/1 -> mpc/1, Scope6/1, Mux3/1
  MATLAB Function10/2(I) -> MATLAB Function7/4(I), MATLAB Function12/4(I)
  MATLAB Function10/5(H) -> MATLAB Function5/1(H), MATLAB Function2/1(H)
  MATLAB Function12/2(bk) -> MATLAB Function2/4(bk), MATLAB Function5/4(bk)
  Demux1/3 -> Mux3/3
  MATLAB Function10/4(Sm) -> MATLAB Function7/7(Sm), MATLAB Function12/2(Sm)
  Memory1/1 -> MATLAB Function1/2(x_k_1)
  MATLAB Function12/1(Cm) -> MATLAB Function2/3(Cm), MATLAB Function5/3(Cm)
  Mux3/1 -> Delay2/1
  Gain3/1 -> Memory/1, MATLAB Function/1(x_k), MATLAB Function7/5(y), MATLAB Function12/5(y)
  Constant6/1 -> MATLAB Function2/6(deltP), MATLAB Function5/6(deltP)
  Delay2/1 -> MATLAB Function2/5(p_last)
  MATLAB Function/1(deltx) -> Scope1/1, MATLAB Function7/3(deltW), MATLAB Function12/3(deltW)
  MATLAB Function10/7(Rk_1) -> MATLAB Function7/1(Rk_1)
  f/1 -> Zero-Order Hold/1
  p/1 -> Zero-Order Hold1/1
  Delay3/1 -> MATLAB Function5/5(p_last)
  MATLAB Function5/1(Uout) -> Scope3/1, Selector/1, Delay3/1
  Selector/1 -> ?
  Zero-Order Hold1/1 -> MATLAB Function1/1(x_k), Memory1/1, Scope/1
  Zero-Order Hold/1 -> Gain3/1
  Constant/1 -> MATLAB Function10/2(Jp)
  Gain/1 -> MATLAB Function10/1(Jw), Scope2/1  "r"
  J/1 -> MATLAB Function10/3(J), Gain1/1
  D/1 -> Sum/2, MATLAB Function10/4(D)
  Sum/1 -> Gain/1
  Gain1/1 -> Sum/1
  Constant2/1 -> ?
  Constant3/1 -> ?
  Constant1/1 -> ?

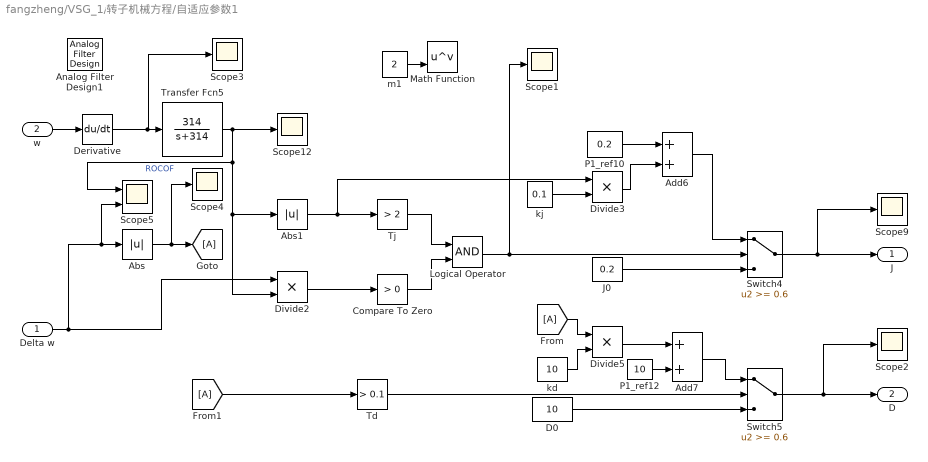
== system fangzheng/VSG_1/转子机械方程/自适应参数1 ==
  Delta w : Inport
  w : Inport  Port=2
  Abs : Abs  SaturateOnIntegerOverflow=off
  Abs1 : Abs  SaturateOnIntegerOverflow=off
  Add6 : Sum
  Add7 : Sum
  Analog Filter Design1 : dspfdesign/Analog Filter Design  method=Butterworth  filttype=Lowpass  N=2  Wlo=50*pi  Whi=80  Rp=2  Rs=40
  Compare To Zero : simulink/Logic and Bit Operations/Compare To Zero  relop=>  OutDataTypeStr=boolean
  D0 : Constant  Value=10
  Derivative : Derivative
  Divide2 : Product  Inputs=**
  Divide3 : Product  Inputs=**
  Divide5 : Product  Inputs=**
  From : From
  From1 : From
  Goto : Goto
  J0 : Constant  Value=0.2
  Logical Operator : Logic  AllPortsSameDT=off  OutDataTypeStr=boolean
  Math Function : Math  Operator=pow  SignedPower=on
  P1_ref10 : Constant  Value=0.2
  P1_ref12 : Constant  Value=10
  Scope{1..4,9,12} (6 alike) : Scope
  Scope5 : Scope  NumInputPorts=2
  Switch4 : Switch  Threshold=0.6  SaturateOnIntegerOverflow=off  InputSameDT=off
  Switch5 : Switch  Threshold=0.6  SaturateOnIntegerOverflow=off  InputSameDT=off
  Td : simulink/Logic and Bit Operations/Compare To Constant  relop=>  const=0.1  OutDataTypeStr=boolean
  Tj : simulink/Logic and Bit Operations/Compare To Constant  relop=>  const=2  OutDataTypeStr=boolean
  Transfer Fcn5 : TransferFcn  Numerator=[314]  Denominator=[1 314]
  kd : Constant  Value=10
  kj : Constant  Value=0.1
  m1 : Constant  Value=2
  J : Outport  VectorParamsAs1DForOutWhenUnconnected=off
  D : Outport  Port=2  VectorParamsAs1DForOutWhenUnconnected=off
  wires:
  Abs1/1 -> Tj/1, Divide3/1
  m1/1 -> Math Function/2
  From1/1 -> Td/1
  Switch5/1 -> D/1, Scope2/1
  Add7/1 -> Switch5/1
  Add6/1 -> Switch4/1
  From/1 -> Divide5/1
  Abs/1 -> Goto/1, Scope4/1
  Transfer Fcn5/1 -> Scope5/1, Abs1/1, Divide2/2, Scope12/1  "ROCOF"
  w/1 -> Derivative/1
  P1_ref12/1 -> Add7/2
  D0/1 -> Switch5/3
  Delta w/1 -> Abs/1, Scope5/2, Divide2/1
  kj/1 -> Divide3/2
  P1_ref10/1 -> Add6/1
  Td/1 -> Switch5/2
  Divide5/1 -> Add7/1
  Divide3/1 -> Add6/2
  J0/1 -> Switch4/3
  kd/1 -> Divide5/2
  Tj/1 -> Logical Operator/1
  Divide2/1 -> Compare To Zero/1
  Compare To Zero/1 -> Logical Operator/2
  Derivative/1 -> Transfer Fcn5/1, Scope3/1
  Switch4/1 -> J/1, Scope9/1
  Logical Operator/1 -> Switch4/2, Scope1/1

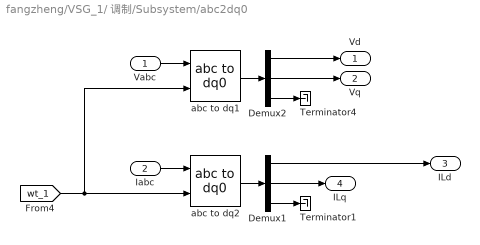
== system fangzheng/VSG_1/ 调制/Subsystem/abc2dq0 ==
  Vabc : Inport
  Iabc : Inport  Port=2
  Demux1 : Demux  Outputs=3
      settings: DisplayOption=none
  Demux2 : Demux  Outputs=3
      settings: DisplayOption=none
  Terminator1 : Terminator
  Terminator4 : Terminator
  abc to dq1 : spsabctodq0Lib/abc to dq0  Alignment=90 degrees behind phase A axis
  abc to dq2 : spsabctodq0Lib/abc to dq0  Alignment=90 degrees behind phase A axis
  Vd : Outport
  Vq : Outport  Port=2
  ILd : Outport  Port=3
  ILq : Outport  Port=4
  wires:
  [wt_1] -> abc to dq2/2, abc to dq1/2
  Vabc/1 -> abc to dq1/1
  abc to dq1/1 -> Demux2/1
  Iabc/1 -> abc to dq2/1
  Demux2/3 -> Terminator4/1
  abc to dq2/1 -> Demux1/1
  Demux1/3 -> Terminator1/1
  Demux1/2 -> ILq/1
  Demux2/1 -> Vd/1
  Demux1/1 -> ILd/1
  Demux2/2 -> Vq/1

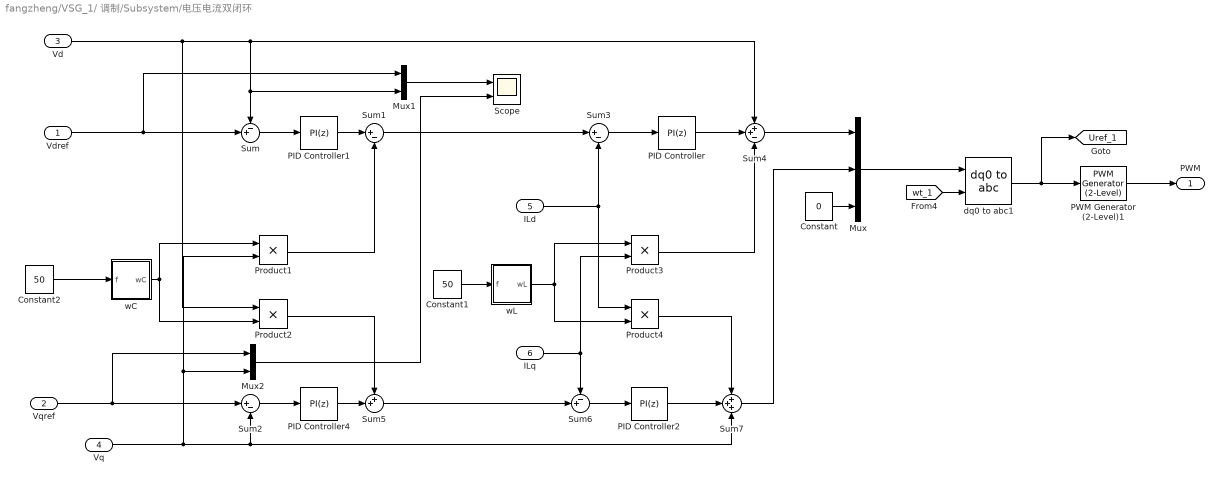
== system fangzheng/VSG_1/ 调制/Subsystem/电压电流双闭环 ==
  Vdref : Inport
  Vqref : Inport  Port=2
  Vd : Inport  Port=3
  Vq : Inport  Port=4
  ILd : Inport  Port=5
  ILq : Inport  Port=6
  Constant : Constant  Value=0
  Constant1 : Constant  Value=50
  Constant2 : Constant  Value=50
  Mux : Mux  Inputs=3
  Mux1 : Mux  Inputs=2
  Mux2 : Mux  Inputs=2
  PID Controller : slpidlib/PID Controller  Controller=PI  Form=Parallel  TimeDomain=Discrete-time  UseExternalTs=off  SampleTime=-1  IntegratorMethod=Forward Euler  FilterMethod=Forward Euler  ControllerParametersSource=internal  P=1  I=10  UseKiTs=off  D=0  N=100  UseFilter=on  TunerSelectOption=Transfer Function Based (PID Tuner App)  InitialConditionSource=internal  InitialConditionForIntegrator=0  InitialConditionForFilter=0  DifferentiatorICPrevScaledInput=0  ExternalReset=none  TrackingMode=off  Kt=1  LimitOutput=off  SatLimitsSource=internal  UpperSaturationLimit=inf  LowerSaturationLimit=-inf  LinearizeAsGain=on  AntiWindupMode=none  Kb=1  LimitIntegrator=off  UpperIntegratorSaturationLimit=inf  LowerIntegratorSaturationLimit=-inf  POutMin=[]  POutMax=[]  IOutMin=[]  IOutMax=[]  DOutMin=[]  DOutMax=[]  NOutMin=[]  NOutMax=[]  SumOutMin=[]  SumOutMax=[]  SaturationOutMin=[]  SaturationOutMax=[]  PParamMin=[]  PParamMax=[]  IParamMin=[]  IParamMax=[]  DParamMin=[]  DParamMax=[]  NParamMin=[]  NParamMax=[]  KbParamMin=[]  KbParamMax=[]  KtParamMin=[]  KtParamMax=[]  KbOutMin=[]  KbOutMax=[]  KtOutMin=[]  KtOutMax=[]  IntegratorOutMin=[]  IntegratorOutMax=[]  FilterOutMin=[]  FilterOutMax=[]  SumI1OutMin=[]  SumI1OutMax=[]  SumI2OutMin=[]  SumI2OutMax=[]  SumI3OutMin=[]  SumI3OutMax=[]  SumI4OutMin=[]  SumI4OutMax=[]  SumDOutMin=[]  SumDOutMax=[]  DifferentiatorOutMin=[]  DifferentiatorOutMax=[]  FilterDiffOutCoefMin=[]  FilterDiffOutCoefMax=[]  ReciprocalOutMin=[]  ReciprocalOutMax=[]  SumDenOutMin=[]  SumDenOutMax=[]  SumNumOutMin=[]  SumNumOutMax=[]  DivideOutMin=[]  DivideOutMax=[]  UdiffTsProdOutMin=[]  UdiffTsProdOutMax=[]  NTsProdOutMin=[]  NTsProdOutMax=[]  UintegralTsProdOutMin=[]  UintegralTsProdOutMax=[]  UngainTsProdOutMin=[]  UngainTsProdOutMax=[]  ClampingZeroOutDataTypeStr=Inherit: Inherit via back propagation  ClampingZeroOutMin=[]  ClampingZeroOutMax=[]  FilterDenConstantOutDataTypeStr=Inherit: Inherit via back propagation  FilterDenConstantOutMin=[]  FilterDenConstantOutMax=[]  PCopyOutDataTypeStr=Inherit: Inherit via back propagation  PCopyOutMin=[]  PCopyOutMax=[]  NCopyOutDataTypeStr=Inherit: Inherit via back propagation  NCopyOutMin=[]  NCopyOutMax=[]  IntegratorContinuousStateAttributes=''  IntegratorStateMustResolveToSignalObject=off  IntegratorRTWStateStorageClass=Auto  FilterContinuousStateAttributes=''  FilterStateMustResolveToSignalObject=off  FilterRTWStateStorageClass=Auto  ParallelPVariant=InternalParameters  IdealPVariant=Disabled  IVariant=InternalParameters  DVariant=Disabled  IntegratorVariant=Discrete  SatVariant=Disabled  AWVariant=Passthrough  PCopyVariant=Disabled  TRVariant=Disabled  FdbkBlocksVariant=Forward  IdealPFdbkVariant=Disabled  SatFdbkVariant=Disabled  DerivativeFilterVariant=Disabled  NVariant=Disabled  NCopyVariant=Disabled_SignalSpec  FilterICVariant=Disabled  IntegratorICVariant=InternalICs  ExternalResetVariant=Disabled  TRSumVariant=Passthrough  SumFdbkVariant=Disabled  SumVariant=Sum_PI  TsampFilterVariant=InternalTs  TsampNgainVariant=Passthrough  TsampIntegralVariant=Disabled_SignalSpec  ExternalSaturationOutDataTypeStr=Inherit: Same as second input
  PID Controller1 : slpidlib/PID Controller  Controller=PI  Form=Parallel  TimeDomain=Discrete-time  UseExternalTs=off  SampleTime=-1  IntegratorMethod=Forward Euler  FilterMethod=Forward Euler  ControllerParametersSource=internal  P=P  I=I  UseKiTs=off  D=30  N=100  UseFilter=on  TunerSelectOption=Transfer Function Based (PID Tuner App)  InitialConditionSource=internal  InitialConditionForIntegrator=0  InitialConditionForFilter=0  DifferentiatorICPrevScaledInput=0  ExternalReset=none  TrackingMode=off  Kt=1  LimitOutput=off  SatLimitsSource=internal  UpperSaturationLimit=inf  LowerSaturationLimit=-inf  LinearizeAsGain=on  AntiWindupMode=none  Kb=1  LimitIntegrator=off  UpperIntegratorSaturationLimit=inf  LowerIntegratorSaturationLimit=-inf  POutMin=[]  POutMax=[]  IOutMin=[]  IOutMax=[]  DOutMin=[]  DOutMax=[]  NOutMin=[]  NOutMax=[]  SumOutMin=[]  SumOutMax=[]  SaturationOutMin=[]  SaturationOutMax=[]  PParamMin=[]  PParamMax=[]  IParamMin=[]  IParamMax=[]  DParamMin=[]  DParamMax=[]  NParamMin=[]  NParamMax=[]  KbParamMin=[]  KbParamMax=[]  KtParamMin=[]  KtParamMax=[]  KbOutMin=[]  KbOutMax=[]  KtOutMin=[]  KtOutMax=[]  IntegratorOutMin=[]  IntegratorOutMax=[]  FilterOutMin=[]  FilterOutMax=[]  SumI1OutMin=[]  SumI1OutMax=[]  SumI2OutMin=[]  SumI2OutMax=[]  SumI3OutMin=[]  SumI3OutMax=[]  SumI4OutMin=[]  SumI4OutMax=[]  SumDOutMin=[]  SumDOutMax=[]  DifferentiatorOutMin=[]  DifferentiatorOutMax=[]  FilterDiffOutCoefMin=[]  FilterDiffOutCoefMax=[]  ReciprocalOutMin=[]  ReciprocalOutMax=[]  SumDenOutMin=[]  SumDenOutMax=[]  SumNumOutMin=[]  SumNumOutMax=[]  DivideOutMin=[]  DivideOutMax=[]  UdiffTsProdOutMin=[]  UdiffTsProdOutMax=[]  NTsProdOutMin=[]  NTsProdOutMax=[]  UintegralTsProdOutMin=[]  UintegralTsProdOutMax=[]  UngainTsProdOutMin=[]  UngainTsProdOutMax=[]  ClampingZeroOutDataTypeStr=Inherit: Inherit via back propagation  ClampingZeroOutMin=[]  ClampingZeroOutMax=[]  FilterDenConstantOutDataTypeStr=Inherit: Inherit via back propagation  FilterDenConstantOutMin=[]  FilterDenConstantOutMax=[]  PCopyOutDataTypeStr=Inherit: Inherit via back propagation  PCopyOutMin=[]  PCopyOutMax=[]  NCopyOutDataTypeStr=Inherit: Inherit via back propagation  NCopyOutMin=[]  NCopyOutMax=[]  IntegratorContinuousStateAttributes=''  IntegratorStateMustResolveToSignalObject=off  IntegratorRTWStateStorageClass=Auto  FilterContinuousStateAttributes=''  FilterStateMustResolveToSignalObject=off  FilterRTWStateStorageClass=Auto  ParallelPVariant=InternalParameters  IdealPVariant=Disabled  IVariant=InternalParameters  DVariant=Disabled  IntegratorVariant=Discrete  SatVariant=Disabled  AWVariant=Passthrough  PCopyVariant=Disabled  TRVariant=Disabled  FdbkBlocksVariant=Forward  IdealPFdbkVariant=Disabled  SatFdbkVariant=Disabled  DerivativeFilterVariant=Disabled  NVariant=Disabled  NCopyVariant=Disabled_SignalSpec  FilterICVariant=Disabled  IntegratorICVariant=InternalICs  ExternalResetVariant=Disabled  TRSumVariant=Passthrough  SumFdbkVariant=Disabled  SumVariant=Sum_PI  TsampFilterVariant=InternalTs  TsampNgainVariant=Passthrough  TsampIntegralVariant=Disabled_SignalSpec  ExternalSaturationOutDataTypeStr=Inherit: Same as second input
  PID Controller2 : slpidlib/PID Controller  Controller=PI  Form=Parallel  TimeDomain=Discrete-time  UseExternalTs=off  SampleTime=-1  IntegratorMethod=Forward Euler  FilterMethod=Forward Euler  ControllerParametersSource=internal  P=1  I=10  UseKiTs=off  D=0  N=100  UseFilter=on  TunerSelectOption=Transfer Function Based (PID Tuner App)  InitialConditionSource=internal  InitialConditionForIntegrator=0  InitialConditionForFilter=0  DifferentiatorICPrevScaledInput=0  ExternalReset=none  TrackingMode=off  Kt=1  LimitOutput=off  SatLimitsSource=internal  UpperSaturationLimit=inf  LowerSaturationLimit=-inf  LinearizeAsGain=on  AntiWindupMode=none  Kb=1  LimitIntegrator=off  UpperIntegratorSaturationLimit=inf  LowerIntegratorSaturationLimit=-inf  POutMin=[]  POutMax=[]  IOutMin=[]  IOutMax=[]  DOutMin=[]  DOutMax=[]  NOutMin=[]  NOutMax=[]  SumOutMin=[]  SumOutMax=[]  SaturationOutMin=[]  SaturationOutMax=[]  PParamMin=[]  PParamMax=[]  IParamMin=[]  IParamMax=[]  DParamMin=[]  DParamMax=[]  NParamMin=[]  NParamMax=[]  KbParamMin=[]  KbParamMax=[]  KtParamMin=[]  KtParamMax=[]  KbOutMin=[]  KbOutMax=[]  KtOutMin=[]  KtOutMax=[]  IntegratorOutMin=[]  IntegratorOutMax=[]  FilterOutMin=[]  FilterOutMax=[]  SumI1OutMin=[]  SumI1OutMax=[]  SumI2OutMin=[]  SumI2OutMax=[]  SumI3OutMin=[]  SumI3OutMax=[]  SumI4OutMin=[]  SumI4OutMax=[]  SumDOutMin=[]  SumDOutMax=[]  DifferentiatorOutMin=[]  DifferentiatorOutMax=[]  FilterDiffOutCoefMin=[]  FilterDiffOutCoefMax=[]  ReciprocalOutMin=[]  ReciprocalOutMax=[]  SumDenOutMin=[]  SumDenOutMax=[]  SumNumOutMin=[]  SumNumOutMax=[]  DivideOutMin=[]  DivideOutMax=[]  UdiffTsProdOutMin=[]  UdiffTsProdOutMax=[]  NTsProdOutMin=[]  NTsProdOutMax=[]  UintegralTsProdOutMin=[]  UintegralTsProdOutMax=[]  UngainTsProdOutMin=[]  UngainTsProdOutMax=[]  ClampingZeroOutDataTypeStr=Inherit: Inherit via back propagation  ClampingZeroOutMin=[]  ClampingZeroOutMax=[]  FilterDenConstantOutDataTypeStr=Inherit: Inherit via back propagation  FilterDenConstantOutMin=[]  FilterDenConstantOutMax=[]  PCopyOutDataTypeStr=Inherit: Inherit via back propagation  PCopyOutMin=[]  PCopyOutMax=[]  NCopyOutDataTypeStr=Inherit: Inherit via back propagation  NCopyOutMin=[]  NCopyOutMax=[]  IntegratorContinuousStateAttributes=''  IntegratorStateMustResolveToSignalObject=off  IntegratorRTWStateStorageClass=Auto  FilterContinuousStateAttributes=''  FilterStateMustResolveToSignalObject=off  FilterRTWStateStorageClass=Auto  ParallelPVariant=InternalParameters  IdealPVariant=Disabled  IVariant=InternalParameters  DVariant=Disabled  IntegratorVariant=Discrete  SatVariant=Disabled  AWVariant=Passthrough  PCopyVariant=Disabled  TRVariant=Disabled  FdbkBlocksVariant=Forward  IdealPFdbkVariant=Disabled  SatFdbkVariant=Disabled  DerivativeFilterVariant=Disabled  NVariant=Disabled  NCopyVariant=Disabled_SignalSpec  FilterICVariant=Disabled  IntegratorICVariant=InternalICs  ExternalResetVariant=Disabled  TRSumVariant=Passthrough  SumFdbkVariant=Disabled  SumVariant=Sum_PI  TsampFilterVariant=InternalTs  TsampNgainVariant=Passthrough  TsampIntegralVariant=Disabled_SignalSpec  ExternalSaturationOutDataTypeStr=Inherit: Same as second input
  PID Controller4 : slpidlib/PID Controller  Controller=PI  Form=Parallel  TimeDomain=Discrete-time  UseExternalTs=off  SampleTime=-1  IntegratorMethod=Forward Euler  FilterMethod=Forward Euler  ControllerParametersSource=internal  P=P  I=I  UseKiTs=off  D=30  N=100  UseFilter=on  TunerSelectOption=Transfer Function Based (PID Tuner App)  InitialConditionSource=internal  InitialConditionForIntegrator=0  InitialConditionForFilter=0  DifferentiatorICPrevScaledInput=0  ExternalReset=none  TrackingMode=off  Kt=1  LimitOutput=off  SatLimitsSource=internal  UpperSaturationLimit=inf  LowerSaturationLimit=-inf  LinearizeAsGain=on  AntiWindupMode=none  Kb=1  LimitIntegrator=off  UpperIntegratorSaturationLimit=inf  LowerIntegratorSaturationLimit=-inf  POutMin=[]  POutMax=[]  IOutMin=[]  IOutMax=[]  DOutMin=[]  DOutMax=[]  NOutMin=[]  NOutMax=[]  SumOutMin=[]  SumOutMax=[]  SaturationOutMin=[]  SaturationOutMax=[]  PParamMin=[]  PParamMax=[]  IParamMin=[]  IParamMax=[]  DParamMin=[]  DParamMax=[]  NParamMin=[]  NParamMax=[]  KbParamMin=[]  KbParamMax=[]  KtParamMin=[]  KtParamMax=[]  KbOutMin=[]  KbOutMax=[]  KtOutMin=[]  KtOutMax=[]  IntegratorOutMin=[]  IntegratorOutMax=[]  FilterOutMin=[]  FilterOutMax=[]  SumI1OutMin=[]  SumI1OutMax=[]  SumI2OutMin=[]  SumI2OutMax=[]  SumI3OutMin=[]  SumI3OutMax=[]  SumI4OutMin=[]  SumI4OutMax=[]  SumDOutMin=[]  SumDOutMax=[]  DifferentiatorOutMin=[]  DifferentiatorOutMax=[]  FilterDiffOutCoefMin=[]  FilterDiffOutCoefMax=[]  ReciprocalOutMin=[]  ReciprocalOutMax=[]  SumDenOutMin=[]  SumDenOutMax=[]  SumNumOutMin=[]  SumNumOutMax=[]  DivideOutMin=[]  DivideOutMax=[]  UdiffTsProdOutMin=[]  UdiffTsProdOutMax=[]  NTsProdOutMin=[]  NTsProdOutMax=[]  UintegralTsProdOutMin=[]  UintegralTsProdOutMax=[]  UngainTsProdOutMin=[]  UngainTsProdOutMax=[]  ClampingZeroOutDataTypeStr=Inherit: Inherit via back propagation  ClampingZeroOutMin=[]  ClampingZeroOutMax=[]  FilterDenConstantOutDataTypeStr=Inherit: Inherit via back propagation  FilterDenConstantOutMin=[]  FilterDenConstantOutMax=[]  PCopyOutDataTypeStr=Inherit: Inherit via back propagation  PCopyOutMin=[]  PCopyOutMax=[]  NCopyOutDataTypeStr=Inherit: Inherit via back propagation  NCopyOutMin=[]  NCopyOutMax=[]  IntegratorContinuousStateAttributes=''  IntegratorStateMustResolveToSignalObject=off  IntegratorRTWStateStorageClass=Auto  FilterContinuousStateAttributes=''  FilterStateMustResolveToSignalObject=off  FilterRTWStateStorageClass=Auto  ParallelPVariant=InternalParameters  IdealPVariant=Disabled  IVariant=InternalParameters  DVariant=Disabled  IntegratorVariant=Discrete  SatVariant=Disabled  AWVariant=Passthrough  PCopyVariant=Disabled  TRVariant=Disabled  FdbkBlocksVariant=Forward  IdealPFdbkVariant=Disabled  SatFdbkVariant=Disabled  DerivativeFilterVariant=Disabled  NVariant=Disabled  NCopyVariant=Disabled_SignalSpec  FilterICVariant=Disabled  IntegratorICVariant=InternalICs  ExternalResetVariant=Disabled  TRSumVariant=Passthrough  SumFdbkVariant=Disabled  SumVariant=Sum_PI  TsampFilterVariant=InternalTs  TsampNgainVariant=Passthrough  TsampIntegralVariant=Disabled_SignalSpec  ExternalSaturationOutDataTypeStr=Inherit: Same as second input
  PWM Generator (2-Level)1 : spsPWMGenerator2LevelLib/PWM Generator (2-Level)  ModulatorType=Three-phase bridge (6 pulses)  ModulatorMode=Unsynchronized  Fc=10e3  Pc=0  nF=27  MinMax="[ -1  1 ]"  SamplingTechnique=Natural  ModulatingSignals=off  m=0.8  Freq=60  Phase=0  Ts=0  ShowCarrierOutport=off
  Product{1..4} (4 alike) : Product
  Scope : Scope  NumInputPorts=2
  Sum : Sum  Inputs=-+|
  Sum1 : Sum  Inputs=|+-
  Sum2 : Sum  Inputs=|+-
  Sum3 : Sum  Inputs=|+-
  Sum4 : Sum  Inputs=++-
  Sum5 : Sum  Inputs=++|
  Sum6 : Sum  Inputs=-+|
  Sum7 : Sum  Inputs=+++
  dq0 to abc1 : spsdq0toabcLib/dq0 to abc  Alignment=90 degrees behind phase A axis
  wC : Subsystem
  wL : Subsystem
  PWM : Outport
  tag scope: Uref_1=global
  wires:
  Mux2/1 -> Scope/2
  Mux1/1 -> Scope/1
  Vqref/1 -> Sum2/1, Mux2/1
  Vdref/1 -> Sum/2, Mux1/1
  Sum5/1 -> Sum6/2
  Sum1/1 -> Sum3/1
  Product1/1 -> Sum1/2
  wC/1(wC) -> Product1/1, Product2/2
  Sum/1 -> PID Controller1/1
  Product2/1 -> Sum5/1
  Constant2/1 -> wC/1(f)
  PID Controller1/1 -> Sum1/1
  Vq/1 -> Sum2/2, Sum7/3, Product1/2, Mux2/2
  Vd/1 -> Product2/1, Sum4/1, Mux1/2, Sum/1
  PID Controller4/1 -> Sum5/2
  Sum2/1 -> PID Controller4/1
  ILq/1 -> Sum6/1, Product3/2
  Sum7/1 -> Mux/2
  Sum4/1 -> Mux/1
  Constant1/1 -> wL/1(f)
  dq0 to abc1/1 -> PWM Generator (2-Level)1/1, [Uref_1]
  Mux/1 -> dq0 to abc1/1
  PWM Generator (2-Level)1/1 -> PWM/1
  PID Controller/1 -> Sum4/2
  Sum3/1 -> PID Controller/1
  Product3/1 -> Sum4/3
  Product4/1 -> Sum7/1
  PID Controller2/1 -> Sum7/2
  Sum6/1 -> PID Controller2/1
  wL/1(wL) -> Product3/1, Product4/2
  ILd/1 -> Product4/1, Sum3/2
  Constant/1 -> Mux/3
  [wt_1] -> dq0 to abc1/2

== system fangzheng/VSG_1/ 调制/Subsystem/电压电流双闭环/wC ==
  f : Inport
  Gain : Gain  Gain=2*pi*Cf*SB/(UB^2)
  wC : Outport
  wires:
  Gain/1 -> wC/1
  f/1 -> Gain/1

== system fangzheng/VSG_1/ 调制/Subsystem/电压电流双闭环/wL ==
  f : Inport
  Constant : Constant  Value=Lf
  Gain : Gain  Gain=2*pi
  Gain1 : Gain  Gain=SB/(UB^2)
  Product : Product
  wL : Outport
  wires:
  Gain1/1 -> wL/1
  f/1 -> Gain/1
  Constant/1 -> Product/1
  Product/1 -> Gain1/1  "WL"
  Gain/1 -> Product/2

== matlab function fangzheng/VSG_1/转子机械方程/Subsystem2/MATLAB Function7 ==
  data: Rk_1 input; SA input; deltW input; I input; y input; Se input; Sm input; deltPe input; Taoy input; G output
function G  = fcn(Rk_1,SA,deltW,I,y,Se,Sm,deltPe,Taoy)
Ep = Rk_1-SA*deltW-I*y-Se*deltPe;
G = 2*Sm.'*(Taoy.'*Taoy)*Ep;
end

== matlab function fangzheng/可编程电源/Embedded MATLAB Function ==
  data: t input; fs input; Kt input; Ua output; U1 input; U5 input; Ub output; Uc output; U7 input; ena output
function [Ua,Ub,Uc,ena] = fcn(t,fs,Kt,U1,U5,U7)
% This block supports the Embedded MATLAB subset.
% See the help menu for details. 

if(t<Kt)
    Ua=U1*sin(2*pi*fs*t);
    Ub=U1*sin(2*pi*fs*t-2*pi/3);
    Uc=U1*sin(2*pi*fs*t+2*pi/3);
    ena=0;
else
    Ua=U1*sin(2*pi*fs*t)+U5*sin(2*pi*fs*5*t)+U7*sin(2*pi*fs*7*t);
    Ub=U1*sin(2*pi*fs*t-2*pi/3)+U5*sin(2*pi*fs*5*t-2*pi/3)+U7*sin(2*pi*fs*7*t-2*pi/3);
    Uc=U1*sin(2*pi*fs*t+2*pi/3)+U5*sin(2*pi*fs*5*t+2*pi/3)+U7*sin(2*pi*fs*7*t+2*pi/3);
    ena=1;
end

== matlab function fangzheng/VSG_1/转子机械方程/Subsystem2/MATLAB Function ==
  data: x_k input; deltx output; x_k_1 input
function deltx = fcn(x_k,x_k_1)

deltx=x_k-x_k_1;

end

== matlab function fangzheng/VSG_1/转子机械方程/Subsystem2/MATLAB Function1 ==
  data: x_k input; deltx output; x_k_1 input
function deltx = fcn(x_k,x_k_1)

deltx=x_k-x_k_1;

end

== matlab function fangzheng/VSG_1/转子机械方程/Subsystem2/MATLAB Function10 ==
  data: SA output; I output; Se output; Sm output; H output; Taoy output; Rk_1 output; Jw input; Jp input; J input; D input
function [SA,I,Se,Sm,H,Taoy,Rk_1] = Init(Jw,Jp,J,D)
%J=0.2;
fn=50;
w0=2*pi*fn;
%D=10;
Ts = 2e-5;
Rk_1=2*pi*fn*ones(5,1);
Taoy=Jw*eye(5);
Taop=Jp*eye(5);
% Pref = 170000;
% if(abs(Pref - Pout)>50000)
%     Taop=0*eye(5);
%     Taoy=20e3*eye(5);
% end


%%%%%%%%%%%%%%%%%预测模型%%%%%%%%%%%%%%%%%%%%%
% 构建离散状态方程
A = exp(-D/J*Ts);
Bm = 9.458984308550447e-08;
%Bm = 1/(J*w0)*integral(@(x)exp(-D/J*x),0,Ts);
Be = -9.458984308550447e-08;
%Be = -1/(J*w0)*integral(@(x)exp(-D/J*x),0,Ts);

% 预测方程
SA = [A;A*A;A*A*A;A*A*A*A;A*A*A*A*A];
I = ones(5,1);


Sm = zeros(5,5);
% for循环，用于构建Phi和Gamma矩阵
Se = zeros(5,1);
Sm(1,1)=Bm;
Se(1,1)=Be;
for i = 2:5
    Se(i) = A*Se(i-1) + Be;
    Sm(i,:) = [A*Sm(i-1,1)+Bm , Sm(i-1,1:4)];
end

H = Sm.'*(Taoy.'*Taoy)*Sm+Taop.'*Taop;

== matlab function fangzheng/VSG_1/转子机械方程/Subsystem2/MATLAB Function12 ==
  data: SA input; Sm input; Cm output; deltW input; I input; y input; Se input; deltPe input; bk output
function [Cm,bk] = fcn(SA,Sm,deltW,I,y,Se,deltPe)
Ymin = 0;
Ymax = 400;
Cm = [-Sm;Sm];
bk = [(SA*deltW+I*y+Se*deltPe)-Ymax;-(SA*deltW+I*y+Se*deltPe)+Ymin];

== matlab function fangzheng/VSG_1/转子机械方程/Subsystem2/MATLAB Function2 ==
  data: H input; Uout output; G input; Cm input; bk input; p_last input; deltP input
function Uout = simpleOptimization(H, G, Cm, bk, p_last, deltP)
    % 定义目标函数 J(x)
    J = @(x) 0.5 * (x(1) + deltP)' * H(1,1) * (x(1) + deltP) + ...
              0.5 * (p_last(3) + deltP)' * H(2,2) * (p_last(3) + deltP) + ...
              0.5 * (p_last(4) + deltP)' * H(3,3) * (p_last(4) + deltP) + ...
              0.5 * (p_last(5) + deltP)' * H(4,4) * (p_last(5) + deltP) + ...
              0.5 * (x(2) + deltP)' * H(5,5) * (x(2) + deltP) - ...
              (G(1) * (x(1) + deltP) + G(3) * (p_last(3) + deltP) + ...
               G(4) * (p_last(4) + deltP) + G(5) * (p_last(5) + deltP) + ...
               G(5) * (x(2) + deltP));

    % 初始化 U0，包含前4个元素为p_last的值，x5为0
    U0 = zeros(2, 1);  % 初始化一个包含 5 个元素的向量
    U0(1) = p_last(1); % 只优化 x1 和 x5
    U0(2) = p_last(5);
    % 设定优化参数
    max_iter = 50000; % 最大迭代次数
    alpha = 0.01; % 学习率
    tolerance = 1e-7; % 收敛容忍度

    Uopt = U0; % 当前优化解
    for iter = 1:max_iter
        % 计算目标函数的梯度
        grad = zeros(2, 1);  % 初始化梯度
        
        % 计算 x1 的梯度
        grad(1) = H(1,1) * (Uopt(1) + deltP) - G(1);
        
        % 计算 x5 的梯度
        grad(2) = H(5,5) * (Uopt(2) + deltP) - G(5);

        % 更新 U
        Unew = Uopt - alpha * grad; 

       %  % 处理约束，确保 Unew 满足线性约束
       %  % 注释掉约束处理部分
       %  for i = 1:length(Cm)
       %      if i <= length(Unew) && Unew(i) < -bk(i)  
       %          Unew(i) = -bk(i); % 应用约束
       %      end
       % end
        
        % 检查目标函数值是否改善
        if J(Unew) < J(Uopt)
            Uopt = Unew; % 更新优化解
        end
        
        % 检查收敛
        if norm(Unew - Uopt) < tolerance
            break;
        end
    end

    % 输出结果，确保输出为列向量
    Uout = [Uopt(1); p_last(3); p_last(4); p_last(5); Uopt(2)];

end

== matlab function fangzheng/VSG_1/转子机械方程/Subsystem2/MATLAB Function5 ==
  data: H input; Uout output; G input; Cm input; bk input; p_last input; deltP input
function Uout = fcn(H,G, Cm, bk, p_last , deltP)

% options = optimoptions('quadprog','Algorithm','active-set'); % 设置算法为'active-set'
% deltPm = quadprog(H,-G,-Cm,-bk,[],[],[],[],[0;0;0;0;0],options); % 调用quadprog，忽略其他约束
%  Pm = deltPm(1,1);

% J = @(x)1/2*[x(1);p_last(3);x(3);p_last(5);x(5)].'*H*[x(1);p_last(3);x(3);p_last(5);x(5)]...
%     -G.'*[x(1);p_last(3);x(3);p_last(5);x(5)];
% U0 = p_last;
% fun=@(x)J(x);
% options = optimoptions('fmincon','Display','iter','Algorithm','sqp');
% [Uopt,fval]= fmincon(fun,U0,-Cm,,[],[],[],[],[],options);
% 
% J = @(x)1/2*[x(1);p_last(3);p_last(4);p_last(5);x(5)].'*H*[x(1);p_last(3);p_last(4);p_last(5);x(5)]...
%     -G.'*[x(1);p_last(3);p_last(4);p_last(5);x(5)];
% U0 = p_last;
% fun=@(x)J(x);
% options = optimoptions('fmincon','Display','iter','Algorithm','sqp');
% [Uopt,fval]= fmincon(fun,U0,-Cm,-bk,[],[],[],[],[],options);

J = @(x)1/2*[x(1)+deltP;x(2)+deltP;x(3)+deltP;x(4)+deltP;x(5)+deltP].'*H*[x(1)+deltP;x(2)+deltP;x(3)+deltP;x(4)+deltP;x(5)+deltP]...
    -G.'*[x(1)+deltP;x(2)+deltP;x(3)+deltP;x(4)+deltP;x(5)+deltP];
U0 = p_last;
fun=@(x)J(x);
options = optimoptions('fmincon','Display','iter','Algorithm','sqp');
[Uopt,fval]= fmincon(fun,U0,-Cm,-bk,[],[],[],[],[],options);
Uout = [Uopt(1);Uopt(2);Uopt(3);Uopt(4);Uopt(5)];
